simulink library "Contact_Forces_Lib"  (R2025b)
settings: Solver=ode45  StartTime=0.0  StopTime=10.0  RelTol=1e-3  EnableMultiTasking=on
undefined symbols (not defined in the file or in its folder): b_contact, custom_param_1, custom_param_2, Extr_Data_Ring, k_contact, l_cone, length_cylinder, length_tube, mu_kinetic, mu_static, pen_exponent, pen_full_damp_F, rad_s_cone, radius_cylinder, radius_tube, v_thr, X, Y, Z
libraries: nesl_utility x197, sm_lib x115, $bdroot x72, simulink x20, fl_lib x4
(part 5 of 12)

== system Contact_Forces_Lib/3D/Sphere to Tube Force ==
  Bus Creator1 : BusCreator  Inputs=3
  Check Active : Subsystem
  Demux : Subsystem
  External Force and Torque SphF : sm_lib/Forces and Torques/External Force and Torque  EnableForceX=on  EnableForceY=on  EnableForceZ=on  EnableForce=off  ForceResolutionFrame=AttachedFrame  EnableTorqueX=off  EnableTorqueY=off  EnableTorqueZ=off  EnableTorque=on  TorqueResolutionFrame=AttachedFrame
  External Force and Torque TubB : sm_lib/Forces and Torques/External Force and Torque  EnableForceX=on  EnableForceY=on  EnableForceZ=on  EnableForce=off  ForceResolutionFrame=AttachedFrame  EnableTorqueX=off  EnableTorqueY=off  EnableTorqueZ=off  EnableTorque=on  TorqueResolutionFrame=AttachedFrame
  Forces : Subsystem
  If1 : If
  Merge : Merge  InitialOutput=0  InputPortOffsets=0
  No Force : Subsystem
  Sensing : Subsystem
  Set Output : Subsystem
  Visual SphF : sm_lib/Body Elements/Spherical Solid  SphereRadius=radius_sphere  SphereRadiusUnits=m  ExportEntireGeometry=off  InertiaType=CalculateFromGeometry  BasedOnType=Density  Density=0  DensityUnits=kg/(m^3)  Mass=1  MassUnits=kg  CenterOfMass=[0 0 0]  CenterOfMassUnits=m  MomentsOfInertia=[1 1 1]  MomentsOfInertiaUnits=kg*m^2  ProductsOfInertia=[0 0 0]  ProductsOfInertiaUnits=kg*m^2  GraphicType=FromGeometry  MarkerShape=Sphere  MarkerSize=10  GraphicVisPropType=SimpleVisualProperties  GraphicDiffuseColor=vis_clr  GraphicOpacity=vis_opc*vis_opc_en  GraphicSpecularColor=[0.5 0.5 0.5 1.0]  GraphicAmbientColor=[0.15 0.15 0.15 1.0]  GraphicEmissiveColor=[0.0 0.0 0.0 1.0]  GraphicShininess=75  DoExposeReferenceFrame=on  SerializedFrames=<Frames/>
  Visual TubB Inner : sm_lib/Body Elements/Extruded Solid  ExtrusionType=General  PolygonNumSides=3  PolygonOuterRadius=1  PolygonOuterRadiusUnits=m  ExportEntireGeometry=off  ExtrusionCrossSection=Extr_Data_Ring(radius_tube-d_tube/2+vis_len_tubBx,radius_tube-d_tube/2,active_angle(1),active_angle(2))  ExtrusionCrossSectionUnits=m  ExportConvexHullGeometry=off  ExtrusionLength=l_tube  ExtrusionLengthUnits=m  InertiaType=CalculateFromGeometry  BasedOnType=Density  Density=0  DensityUnits=kg/(m^3)  Mass=1  MassUnits=kg  CenterOfMass=[0 0 0]  CenterOfMassUnits=m  MomentsOfInertia=[1 1 1]  MomentsOfInertiaUnits=kg*m^2  ProductsOfInertia=[0 0 0]  ProductsOfInertiaUnits=kg*m^2  GraphicType=FromGeometry  MarkerShape=Sphere  MarkerSize=10  GraphicVisPropType=SimpleVisualProperties  GraphicDiffuseColor=vis_clr  GraphicOpacity=vis_opc*vis_opc_en  GraphicSpecularColor=[0.5 0.5 0.5 1.0]  GraphicAmbientColor=[0.15 0.15 0.15 1.0]  GraphicEmissiveColor=[0.0 0.0 0.0 1.0]  GraphicShininess=75  DoExposeReferenceFrame=on  SerializedFrames=<Frames/>
  Visual TubB Outer : sm_lib/Body Elements/Extruded Solid  ExtrusionType=General  PolygonNumSides=3  PolygonOuterRadius=1  PolygonOuterRadiusUnits=m  ExportEntireGeometry=off  ExtrusionCrossSection=Extr_Data_Ring(radius_tube+d_tube/2,radius_tube+d_tube/2-vis_len_tubBx,active_angle(1),active_angle(2))  ExtrusionCrossSectionUnits=m  ExportConvexHullGeometry=off  ExtrusionLength=l_tube  ExtrusionLengthUnits=m  InertiaType=CalculateFromGeometry  BasedOnType=Density  Density=0  DensityUnits=kg/(m^3)  Mass=1  MassUnits=kg  CenterOfMass=[0 0 0]  CenterOfMassUnits=m  MomentsOfInertia=[1 1 1]  MomentsOfInertiaUnits=kg*m^2  ProductsOfInertia=[0 0 0]  ProductsOfInertiaUnits=kg*m^2  GraphicType=FromGeometry  MarkerShape=Sphere  MarkerSize=10  GraphicVisPropType=SimpleVisualProperties  GraphicDiffuseColor=vis_clr  GraphicOpacity=vis_opc*vis_opc_en  GraphicSpecularColor=[0.5 0.5 0.5 1.0]  GraphicAmbientColor=[0.15 0.15 0.15 1.0]  GraphicEmissiveColor=[0.0 0.0 0.0 1.0]  GraphicShininess=75  DoExposeReferenceFrame=on  SerializedFrames=<Frames/>
  SphF : PMIOPort  Tag=PMCPort  Side=Left
  TubB : PMIOPort  Tag=PMCPort  Port=2  Side=Right
  Out : Outport  VectorParamsAs1DForOutWhenUnconnected=off
  wires:
  Sensing/10(wyf) -> Forces/10(wyf)
  Sensing/9(wxf) -> Forces/9(wxf)
  Sensing/8(vzf) -> Forces/8(vzf)
  Sensing/1(z) -> Check Active/1(z), Forces/1(z)
  Merge/1 -> Demux/1(Frc)  "Total Force"
  Sensing/6(wzf) -> Forces/6(wzf)
  Sensing/3(vrad) -> Forces/3(vrad), Bus Creator1/2  "vrad"
  Sensing/4(azm) -> Check Active/2(azm), Forces/4(azm), Bus Creator1/3  "azm"
  If1/2 -> No Force/Action
  If1/1 -> Forces/Action
  No Force/1(F) -> Merge/1
  Forces/1(Frc) -> Merge/2
  Sensing/7(R) -> Forces/7(R)
  Sensing/2(rad) -> Forces/2(rad), Bus Creator1/1  "rad"
  Sensing/5(vazm) -> Forces/5(vazm)
  Forces/2(Out) -> Set Output/1(Frc)
  Bus Creator1/1 -> Set Output/3(FrameSep)  "Frame Sep"
  Set Output/1(Out) -> Out/1
  Check Active/1(En) -> Set Output/2(En), If1/1
  connections:
  Demux/RConn8 -- External Force and Torque TubB/LConn4
  Demux/RConn7 -- External Force and Torque TubB/LConn3
  Demux/RConn6 -- External Force and Torque TubB/LConn2
  Demux/RConn5 -- External Force and Torque TubB/LConn1
  Demux/RConn4 -- External Force and Torque SphF/LConn4
  Demux/RConn3 -- External Force and Torque SphF/LConn3
  Demux/RConn2 -- External Force and Torque SphF/LConn2
  Demux/RConn1 -- External Force and Torque SphF/LConn1
  External Force and Torque SphF/RConn1 -- Visual SphF/RConn1 -- SphF/RConn1 -- Sensing/LConn1
  Visual TubB Outer/RConn1 -- Visual TubB Inner/RConn1 -- TubB/RConn1 -- Sensing/LConn2 -- External Force and Torque TubB/RConn1

== system Contact_Forces_Lib/3D/Sphere to Tube Force Enabled ==
  In : Inport
  Bus Creator1 : BusCreator  Inputs=3
  Bus Selector1 : BusSelector  OutputSignals=Enable
  Check Active : Subsystem
  Demux : Subsystem
  External Force and Torque SphF : sm_lib/Forces and Torques/External Force and Torque  EnableForceX=on  EnableForceY=on  EnableForceZ=on  EnableForce=off  ForceResolutionFrame=AttachedFrame  EnableTorqueX=off  EnableTorqueY=off  EnableTorqueZ=off  EnableTorque=on  TorqueResolutionFrame=AttachedFrame
  External Force and Torque TubB : sm_lib/Forces and Torques/External Force and Torque  EnableForceX=on  EnableForceY=on  EnableForceZ=on  EnableForce=off  ForceResolutionFrame=AttachedFrame  EnableTorqueX=off  EnableTorqueY=off  EnableTorqueZ=off  EnableTorque=on  TorqueResolutionFrame=AttachedFrame
  Forces : Subsystem
  If1 : If  NumInputs=2  IfExpression=(u1 > 0 & u2>0)
  In1 : InportShadow
  Merge : Merge  InitialOutput=0  InputPortOffsets=0
  No Force : Subsystem
  Sensing : Subsystem
  Set Output : Subsystem
  Visual SphF : sm_lib/Body Elements/Spherical Solid  SphereRadius=radius_sphere  SphereRadiusUnits=m  ExportEntireGeometry=off  InertiaType=CalculateFromGeometry  BasedOnType=Density  Density=0  DensityUnits=kg/(m^3)  Mass=1  MassUnits=kg  CenterOfMass=[0 0 0]  CenterOfMassUnits=m  MomentsOfInertia=[1 1 1]  MomentsOfInertiaUnits=kg*m^2  ProductsOfInertia=[0 0 0]  ProductsOfInertiaUnits=kg*m^2  GraphicType=FromGeometry  MarkerShape=Sphere  MarkerSize=10  GraphicVisPropType=SimpleVisualProperties  GraphicDiffuseColor=vis_clr  GraphicOpacity=vis_opc*vis_opc_en  GraphicSpecularColor=[0.5 0.5 0.5 1.0]  GraphicAmbientColor=[0.15 0.15 0.15 1.0]  GraphicEmissiveColor=[0.0 0.0 0.0 1.0]  GraphicShininess=75  DoExposeReferenceFrame=on  SerializedFrames=<Frames/>
  Visual TubB Inner : sm_lib/Body Elements/Extruded Solid  ExtrusionType=General  PolygonNumSides=3  PolygonOuterRadius=1  PolygonOuterRadiusUnits=m  ExportEntireGeometry=off  ExtrusionCrossSection=Extr_Data_Ring(radius_tube-d_tube/2+vis_len_tubBx,radius_tube-d_tube/2,active_angle(1),active_angle(2))  ExtrusionCrossSectionUnits=m  ExportConvexHullGeometry=off  ExtrusionLength=l_tube  ExtrusionLengthUnits=m  InertiaType=CalculateFromGeometry  BasedOnType=Density  Density=0  DensityUnits=kg/(m^3)  Mass=1  MassUnits=kg  CenterOfMass=[0 0 0]  CenterOfMassUnits=m  MomentsOfInertia=[1 1 1]  MomentsOfInertiaUnits=kg*m^2  ProductsOfInertia=[0 0 0]  ProductsOfInertiaUnits=kg*m^2  GraphicType=FromGeometry  MarkerShape=Sphere  MarkerSize=10  GraphicVisPropType=SimpleVisualProperties  GraphicDiffuseColor=vis_clr  GraphicOpacity=vis_opc*vis_opc_en  GraphicSpecularColor=[0.5 0.5 0.5 1.0]  GraphicAmbientColor=[0.15 0.15 0.15 1.0]  GraphicEmissiveColor=[0.0 0.0 0.0 1.0]  GraphicShininess=75  DoExposeReferenceFrame=on  SerializedFrames=<Frames/>
  Visual TubB Outer : sm_lib/Body Elements/Extruded Solid  ExtrusionType=General  PolygonNumSides=3  PolygonOuterRadius=1  PolygonOuterRadiusUnits=m  ExportEntireGeometry=off  ExtrusionCrossSection=Extr_Data_Ring(radius_tube+d_tube/2,radius_tube+d_tube/2-vis_len_tubBx,active_angle(1),active_angle(2))  ExtrusionCrossSectionUnits=m  ExportConvexHullGeometry=off  ExtrusionLength=l_tube  ExtrusionLengthUnits=m  InertiaType=CalculateFromGeometry  BasedOnType=Density  Density=0  DensityUnits=kg/(m^3)  Mass=1  MassUnits=kg  CenterOfMass=[0 0 0]  CenterOfMassUnits=m  MomentsOfInertia=[1 1 1]  MomentsOfInertiaUnits=kg*m^2  ProductsOfInertia=[0 0 0]  ProductsOfInertiaUnits=kg*m^2  GraphicType=FromGeometry  MarkerShape=Sphere  MarkerSize=10  GraphicVisPropType=SimpleVisualProperties  GraphicDiffuseColor=vis_clr  GraphicOpacity=vis_opc*vis_opc_en  GraphicSpecularColor=[0.5 0.5 0.5 1.0]  GraphicAmbientColor=[0.15 0.15 0.15 1.0]  GraphicEmissiveColor=[0.0 0.0 0.0 1.0]  GraphicShininess=75  DoExposeReferenceFrame=on  SerializedFrames=<Frames/>
  SphF : PMIOPort  Tag=PMCPort  Side=Left
  TubB : PMIOPort  Tag=PMCPort  Port=2  Side=Right
  Out : Outport  VectorParamsAs1DForOutWhenUnconnected=off
  wires:
  In1/1 -> Sensing/1(In)
  Bus Selector1/1 -> If1/1  "<Enable>"
  In/1 -> Bus Selector1/1
  Sensing/10(wyf) -> Forces/10(wyf)
  Sensing/9(wxf) -> Forces/9(wxf)
  Sensing/8(vzf) -> Forces/8(vzf)
  Sensing/1(z) -> Check Active/1(z), Forces/1(z)
  Merge/1 -> Demux/1(Frc)  "Total Force"
  Sensing/6(wzf) -> Forces/6(wzf)
  Sensing/3(vrad) -> Forces/3(vrad), Bus Creator1/2  "vrad"
  Sensing/4(azm) -> Check Active/2(azm), Forces/4(azm), Bus Creator1/3  "azm"
  If1/2 -> No Force/Action
  If1/1 -> Forces/Action
  No Force/1(F) -> Merge/1
  Forces/1(Frc) -> Merge/2
  Sensing/7(R) -> Forces/7(R)
  Sensing/2(rad) -> Forces/2(rad), Bus Creator1/1  "rad"
  Sensing/5(vazm) -> Forces/5(vazm)
  Forces/2(Out) -> Set Output/1(Frc)
  Bus Creator1/1 -> Set Output/3(FrameSep)  "Frame Sep"
  Set Output/1(Out) -> Out/1
  Check Active/1(En) -> If1/2, Set Output/2(En)
  connections:
  Demux/RConn8 -- External Force and Torque TubB/LConn4
  Demux/RConn7 -- External Force and Torque TubB/LConn3
  Demux/RConn6 -- External Force and Torque TubB/LConn2
  Demux/RConn5 -- External Force and Torque TubB/LConn1
  Demux/RConn4 -- External Force and Torque SphF/LConn4
  Demux/RConn3 -- External Force and Torque SphF/LConn3
  Demux/RConn2 -- External Force and Torque SphF/LConn2
  Demux/RConn1 -- External Force and Torque SphF/LConn1
  SphF/RConn1 -- External Force and Torque SphF/RConn1 -- Visual SphF/RConn1 -- Sensing/LConn1
  Visual TubB Outer/RConn1 -- Visual TubB Inner/RConn1 -- Sensing/LConn2 -- TubB/RConn1 -- External Force and Torque TubB/RConn1

== system Contact_Forces_Lib/Constraints/Cam Roller Constraint ==
  Cam : sm_lib/Body Elements/Extruded Solid  ExtrusionType=General  PolygonNumSides=3  PolygonOuterRadius=1  PolygonOuterRadiusUnits=m  ExportEntireGeometry=off  ExtrusionCrossSection=cam_extr_data  ExtrusionCrossSectionUnits=m  ExportConvexHullGeometry=off  ExtrusionLength=cam_thk  ExtrusionLengthUnits=m  InertiaType=CalculateFromGeometry  BasedOnType=Density  Density=cam_rho  DensityUnits=kg/m^3  Mass=1  MassUnits=kg  CenterOfMass=[0 0 0]  CenterOfMassUnits=m  MomentsOfInertia=[1 1 1]  MomentsOfInertiaUnits=kg*m^2  ProductsOfInertia=[1 1 1]  ProductsOfInertiaUnits=kg*m^2  GraphicType=FromGeometry  MarkerShape=Sphere  MarkerSize=10  GraphicVisPropType=SimpleVisualProperties  GraphicDiffuseColor=cam_clr  GraphicOpacity=cam_opc  GraphicSpecularColor=[0.5 0.5 0.5 1.0]  GraphicAmbientColor=[0.15 0.15 0.15 1.0]  GraphicEmissiveColor=[0.0 0.0 0.0 1.0]  GraphicShininess=75  DoExposeReferenceFrame=on  SerializedFrames=<Frames/>
  Point on Curve Constraint : sm_lib/Constraints/Point on Curve Constraint  WrenchDir=FollowerOnBase  WrenchFrame=BaseFrame  SenseForce=off  SenseTorque=off
  Roller : sm_lib/Body Elements/Cylindrical Solid  CylinderRadius=roller_rad  CylinderRadiusUnits=m  CylinderLength=roller_thk  CylinderLengthUnits=m  ExportEntireGeometry=off  InertiaType=CalculateFromGeometry  BasedOnType=Density  Density=roller_rho  DensityUnits=kg/m^3  Mass=1  MassUnits=kg  CenterOfMass=[0 0 0]  CenterOfMassUnits=m  MomentsOfInertia=[1 1 1]  MomentsOfInertiaUnits=kg*m^2  ProductsOfInertia=[1 1 1]  ProductsOfInertiaUnits=kg*m^2  GraphicType=FromGeometry  MarkerShape=Sphere  MarkerSize=10  GraphicVisPropType=SimpleVisualProperties  GraphicDiffuseColor=roller_clr  GraphicOpacity=roller_opc  GraphicSpecularColor=[0.5 0.5 0.5 1.0]  GraphicAmbientColor=[0.15 0.15 0.15 1.0]  GraphicEmissiveColor=[0.0 0.0 0.0 1.0]  GraphicShininess=75  DoExposeReferenceFrame=on  SerializedFrames=<Frames/>
  Spline : sm_lib/Curves and Surfaces/Spline  DataPoints=roller_curve  DataPointsUnits=m  EndConditionType=Closed  GraphicType=FromGeometry  MarkerShape=Sphere  MarkerSize=10  GraphicVisPropType=SimpleVisualProperties  GraphicDiffuseColor=roller_curve_clr  GraphicOpacity=roller_curve_opc  GraphicSpecularColor=[0.5 0.5 0.5 1.0]  GraphicAmbientColor=[0.15 0.15 0.15 1.0]  GraphicEmissiveColor=[0.0 0.0 0.0 1.0]  GraphicShininess=75
  C : PMIOPort  Side=Right
  R : PMIOPort  Port=2  Side=Left
  connections:
  C/RConn1 -- Cam/RConn1 -- Spline/LConn1
  Spline/RConn1 -- Point on Curve Constraint/LConn1
  Point on Curve Constraint/RConn1 -- R/RConn1 -- Roller/RConn1

== system Contact_Forces_Lib/Force Law/Custom ==
  note: Implement your own custom force law in this subsystem.
      | To use it in the contact force models,
      | set the parameter "Force Law" to "Custom".
  Pen : Inport
  Pen Vel : Inport  Port=2
  Abs : Abs  ZeroCross=off  SaturateOnIntegerOverflow=off
  Gain1 : Gain  Gain=k_pen  Multiplication=Matrix(K*u)  SaturateOnIntegerOverflow=on  OutDataTypeStr=Inherit: Same as input  ParamDataTypeStr=Inherit: Same as input
  Gain2 : Gain  Gain=-b_penvel  Multiplication=Matrix(K*u)  SaturateOnIntegerOverflow=on  OutDataTypeStr=Inherit: Same as input  ParamDataTypeStr=Inherit: Same as input
  Product : Product  RndMeth=Zero
  Saturation : Saturate  UpperLimit=Inf  LowerLimit=0  ZeroCross=off
  Sign : Signum  ZeroCross=off
  Spr F : Outport  VectorParamsAs1DForOutWhenUnconnected=off
  Damp F : Outport  Port=2  VectorParamsAs1DForOutWhenUnconnected=off
  wires:
  Gain1/1 -> Spr F/1  "Stiffness_Force"
  Gain2/1 -> Product/2  "Damping_Force"
  Pen Vel/1 -> Saturation/1  "Pen Vel"
  Sign/1 -> Abs/1
  Product/1 -> Damp F/1  "Damping_Force"
  Abs/1 -> Product/1  "Damping_Force_Enable"
  Pen/1 -> Gain1/1, Sign/1  "Penetration"
  Saturation/1 -> Gain2/1

== system Contact_Forces_Lib/Force Law/Linear ==
  Pen : Inport
  Pen Vel : Inport  Port=2
  Abs : Abs  ZeroCross=off  SaturateOnIntegerOverflow=off
  Gain1 : Gain  Gain=k_pen  Multiplication=Matrix(K*u)  SaturateOnIntegerOverflow=on  OutDataTypeStr=Inherit: Same as input  ParamDataTypeStr=Inherit: Same as input
  Gain2 : Gain  Gain=-b_penvel  Multiplication=Matrix(K*u)  SaturateOnIntegerOverflow=on  OutDataTypeStr=Inherit: Same as input  ParamDataTypeStr=Inherit: Same as input
  Product : Product  RndMeth=Zero
  Saturation : Saturate  UpperLimit=Inf  LowerLimit=0  ZeroCross=off
  Sign : Signum  ZeroCross=off
  Spr F : Outport  VectorParamsAs1DForOutWhenUnconnected=off
  Damp F : Outport  Port=2  VectorParamsAs1DForOutWhenUnconnected=off
  wires:
  Gain1/1 -> Spr F/1  "Stiffness_Force"
  Gain2/1 -> Product/2  "Damping_Force"
  Pen Vel/1 -> Saturation/1  "Pen Vel"
  Sign/1 -> Abs/1
  Product/1 -> Damp F/1  "Damping_Force"
  Abs/1 -> Product/1  "Damping_Force_Enable"
  Pen/1 -> Gain1/1, Sign/1  "Penetration"
  Saturation/1 -> Gain2/1

== system Contact_Forces_Lib/Force Law/Nonlinear ==
  Pen : Inport
  Pen Vel : Inport  Port=2
  Constant : Constant  Value=pen_exp
  Gain1 : Gain  Gain=k_pen  Multiplication=Matrix(K*u)  SaturateOnIntegerOverflow=on  OutDataTypeStr=Inherit: Same as input  ParamDataTypeStr=Inherit: Same as input
  Gain2 : Gain  Gain=-b_penvel  Multiplication=Matrix(K*u)  SaturateOnIntegerOverflow=on  OutDataTypeStr=Inherit: Same as input  ParamDataTypeStr=Inherit: Same as input
  Math Function : Math  Operator=pow  SignedPower=on
  Product1 : Product  RndMeth=Zero
  Saturation : Saturate  UpperLimit=Inf  LowerLimit=0  ZeroCross=off
  Smoothstep : Subsystem  mask{min_out=0, max_out=1, step_start=0, step_finish=pen_full_damping}
      mask prompts: min_out "Minimum output"; max_out "Maximum output"; step_start "Start Step"; step_finish "Finish Step"
  Spr F : Outport  VectorParamsAs1DForOutWhenUnconnected=off
  Damp F : Outport  Port=2  VectorParamsAs1DForOutWhenUnconnected=off
  wires:
  Gain1/1 -> Spr F/1  "Stiffness_Force"
  Pen Vel/1 -> Saturation/1  "Penetration_Velocity"
  Pen/1 -> Smoothstep/1(In1), Math Function/1  "Penetration"
  Math Function/1 -> Gain1/1
  Constant/1 -> Math Function/2
  Gain2/1 -> Product1/2  "Damping_Force"
  Smoothstep/1(Out1) -> Product1/1  "Damping_Enable"
  Product1/1 -> Damp F/1
  Saturation/1 -> Gain2/1

== system Contact_Forces_Lib/Friction Law/None ==
  Fn : Inport
  v : Inport  Port=2
  Constant : Constant  Value=0
  Terminator : Terminator
  Terminator1 : Terminator
  Ff : Outport  VectorParamsAs1DForOutWhenUnconnected=off
  wires:
  Fn/1 -> Terminator1/1  "Normal_Force"
  v/1 -> Terminator/1  "Velocity"
  Constant/1 -> Ff/1  "Friction_Force"

== system Contact_Forces_Lib/Friction Law/Stick-Slip C  ==
  Fn : Inport
  v : Inport  Port=2
  Coefficient of Friction vs Velocity : Lookup_n-D  NumberOfTableDimensions=1  BreakpointsForDimension1=[-3 -1.5 -1 1 1.5 3]*vth  Table="[-muk -muk -mus mus  muk muk]"  InternalRulePriority=Speed
  Gain2 : Gain  Multiplication=Matrix(K*u)  SaturateOnIntegerOverflow=on  OutDataTypeStr=Inherit: Same as input  ParamDataTypeStr=Inherit: Same as input
  Product : Product  RndMeth=Zero
  Ff : Outport  VectorParamsAs1DForOutWhenUnconnected=off
  wires:
  Gain2/1 -> Ff/1  "Friction_Force"
  Product/1 -> Gain2/1
  v/1 -> Coefficient of Friction vs Velocity/1  "Velocity"
  Coefficient of Friction vs Velocity/1 -> Product/1
  Fn/1 -> Product/2  "Normal_Force"

== system Contact_Forces_Lib/Friction Utilities/Stick-Slip Friction 1D ==
  Abs : Abs  ZeroCross=off  SaturateOnIntegerOverflow=off
  Gain : Gain  Gain=-1
  Lag Filter : Subsystem  mask(First-order lag supporting vector signals){b=filt_const, x_initial=0}
      mask prompts: b "Filter time constant"; x_initial "Initial output"
      mask help: Models a lag of the form 1/(b*s+1) where s is the Laplace operator.
  PS-Simulink Converter : nesl_utility/PS-Simulink Converter  PhysicalDomain=network_engine_domain  SubClassName=ps_output  LeftPortType=input  RightPortType=output  PseudoPeriodic=off  Frequencies=[]  VectorFormat=1-D array  Unit=1  AffineConversion=off
  PS-Simulink Converter1 : nesl_utility/PS-Simulink Converter  PhysicalDomain=network_engine_domain  SubClassName=ps_output  LeftPortType=input  RightPortType=output  PseudoPeriodic=off  Frequencies=[]  VectorFormat=1-D array  Unit=1  AffineConversion=off
  Product : $bdroot/Friction Utilities/Utilities/Product  SystemSampleTime=-1  LabelModeActiveChoice=FcConst  VariantActivationTime=update diagram  EmptyChoice=off  PassThrough=off  PassThroughVariantControl=(default)  EmptyChoiceVariantControl=(default)  AllowFlexibleInterface=on  Latency=0  AutoFrameSizeCalculation=off
  Selector : Selector  InputPortWidth=3  IndexOptions=Index vector (dialog)  Indices=[1]  OutputSizes=1
  Simulink-PS Converter1 : nesl_utility/Simulink-PS Converter  PhysicalDomain=network_engine_domain  SubClassName=ps_input  LeftPortType=input  RightPortType=output  PseudoPeriodic=off  Frequencies=[]  NoiseDistribution=none  NoiseParameters=[]  Unit=1  AffineConversion=off  FilteringAndDerivatives=zero  SimscapeFilterOrder=2  InputFilterTimeConstant=0.005  UdotUserProvided=1
  "Stick-Slip C " : $bdroot/Friction Law/Stick-Slip C   VariantControl=Stick_Slip_C  muk=mu_kinetic  mus=mu_static  vth=vel_th
  Vectorize : Gain  Gain=[1 1 1]
  f : PMIOPort  Side=Right
  Fc : PMIOPort  Port=2  Side=Left
  v : PMIOPort  Port=3  Side=Left
  wires:
  Gain/1 -> "Stick-Slip C "/1
  Abs/1 -> Gain/1
  Vectorize/1 -> Selector/1
  PS-Simulink Converter/1 -> "Stick-Slip C "/2
  PS-Simulink Converter1/1 -> Vectorize/1
  "Stick-Slip C "/1 -> Lag Filter/1(In)
  Selector/1 -> Abs/1
  Lag Filter/1(Out) -> Simulink-PS Converter1/1
  connections:
  v/RConn1 -- PS-Simulink Converter/LConn1 -- Product/RConn2
  Fc/RConn1 -- PS-Simulink Converter1/LConn1 -- Product/RConn1
  Simulink-PS Converter1/RConn1 -- f/RConn1

== system Contact_Forces_Lib/Friction Utilities/Utilities ==
  Product : Subsystem  Variant=on  VariantControlMode=label  LabelModeActiveChoice=FcConst

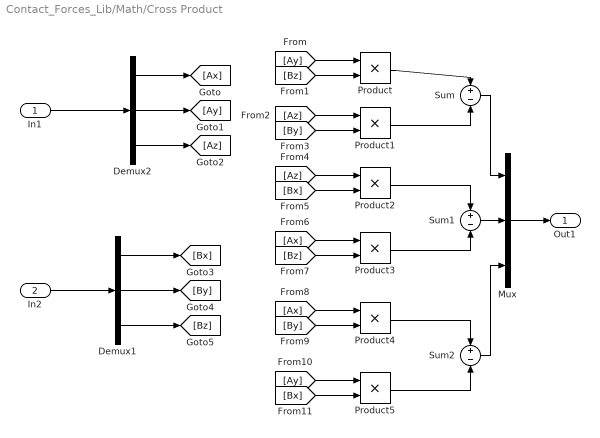
== system Contact_Forces_Lib/Math/Cross Product ==
  In1 : Inport
  In2 : Inport  Port=2
  Demux1 : Demux  Outputs=3
  Demux2 : Demux  Outputs=3
  Mux : Mux  Inputs=3
  Product{,1..5} (6 alike) : Product
  Sum : Sum  Inputs=+|-
  Sum1 : Sum  Inputs=+|-
  Sum2 : Sum  Inputs=+|-
  Out1 : Outport  VectorParamsAs1DForOutWhenUnconnected=off
  wires:
  [Bx] -> Product5/2
  [Ay] -> Product5/1
  [By] -> Product4/2
  [Ax] -> Product4/1
  [Bz] -> Product3/2
  [Ax] -> Product3/1
  [Bx] -> Product2/2
  [Az] -> Product2/1
  [By] -> Product1/2
  [Az] -> Product1/1
  [Bz] -> Product/2
  [Ay] -> Product/1
  Demux1/3 -> [Bz]
  Demux1/2 -> [By]
  Demux1/1 -> [Bx]
  Demux2/3 -> [Az]
  Demux2/2 -> [Ay]
  Demux2/1 -> [Ax]
  In1/1 -> Demux2/1
  Sum2/1 -> Mux/3
  Sum/1 -> Mux/1
  Sum1/1 -> Mux/2
  Product5/1 -> Sum2/2
  Product4/1 -> Sum2/1
  Product3/1 -> Sum1/2
  Product2/1 -> Sum1/1
  Product/1 -> Sum/1
  Product1/1 -> Sum/2
  Mux/1 -> Out1/1
  In2/1 -> Demux1/1

== system Contact_Forces_Lib/Other Forces/Attraction Force ==
  Pen : Inport
  Pen Vel : Inport  Port=2
  Abs : Abs  SaturateOnIntegerOverflow=off
  Dead Zone Center : DeadZone  LowerValue=-inf  UpperValue=0
  Dead Zone Radius : Constant  Value=max_sep*deadzone
  Enable Stiffness Force : Product  RndMeth=Zero
  Gain1 : Gain  Gain=k_pen  Multiplication=Matrix(K*u)  SaturateOnIntegerOverflow=on  OutDataTypeStr=Inherit: Same as input  ParamDataTypeStr=Inherit: Same as input
  Gain2 : Gain  Gain=-b_penvel  Multiplication=Matrix(K*u)  SaturateOnIntegerOverflow=on  OutDataTypeStr=Inherit: Same as input  ParamDataTypeStr=Inherit: Same as input
  Gain3 : Gain  Gain=1e2  Multiplication=Matrix(K*u)  SaturateOnIntegerOverflow=on  OutDataTypeStr=Inherit: Same as input  ParamDataTypeStr=Inherit: Same as input
  Product : Product  RndMeth=Zero
  Sum1 : Sum  Inputs=|-+
  Spr Force : Outport  VectorParamsAs1DForOutWhenUnconnected=off
  Damp Force : Outport  Port=2  VectorParamsAs1DForOutWhenUnconnected=off
  wires:
  Enable Stiffness Force/1 -> Spr Force/1
  Gain1/1 -> Enable Stiffness Force/1  "Stiffness_Force"
  Dead Zone Center/1 -> Enable Stiffness Force/2
  Sum1/1 -> Dead Zone Center/1
  Dead Zone Radius/1 -> Sum1/2
  Pen/1 -> Sum1/1, Gain1/1, Gain3/1  "Penetration"
  Abs/1 -> Product/1  "Damping_Force_Enable"
  Product/1 -> Damp Force/1  "Damping_Force"
  Gain3/1 -> Abs/1
  Pen Vel/1 -> Gain2/1  "Penetration_Velocity"
  Gain2/1 -> Product/2  "Damping_Force"

== system Contact_Forces_Lib/2D/Circle to Circle Force/Calculate Penetration ==
  rad : Inport
  vrad : Inport  Port=2
  Constant : Constant  Value=cirF_rad+cirB_rad
  Dead Zone : DeadZone  LowerValue=-inf  UpperValue=0
  Gain2 : Gain  Gain=-1
  Sum1 : Sum  Inputs=+-
  Pen : Outport  VectorParamsAs1DForOutWhenUnconnected=off
  Pen Vel : Outport  Port=2  VectorParamsAs1DForOutWhenUnconnected=off
  wires:
  rad/1 -> Sum1/2
  Constant/1 -> Sum1/1
  Sum1/1 -> Dead Zone/1
  Dead Zone/1 -> Pen/1
  Gain2/1 -> Pen Vel/1
  vrad/1 -> Gain2/1

== system Contact_Forces_Lib/2D/Circle to Circle Force/Ff ==
  Fn : Inport
  azm : Inport  Port=2
  Pen : Inport  Port=3
  rad : Inport  Port=4
  R : Inport  Port=5
  wz : Inport  Port=6
  vazm : Inport  Port=7
  "Calculate vRel at CP " : Subsystem
  Friction Law : $bdroot/Friction Law  SystemSampleTime=-1  LabelModeActiveChoice=None  VariantActivationTime=update diagram  EmptyChoice=off  PassThrough=off  PassThroughVariantControl=(default)  EmptyChoiceVariantControl=(default)  AllowFlexibleInterface=on  Latency=0  AutoFrameSizeCalculation=off
  Resolve Ff : Subsystem
  FxCirF : Outport  VectorParamsAs1DForOutWhenUnconnected=off
  FyCirF : Outport  Port=2  VectorParamsAs1DForOutWhenUnconnected=off
  FxCirB : Outport  Port=3  VectorParamsAs1DForOutWhenUnconnected=off
  FyCirB : Outport  Port=4  VectorParamsAs1DForOutWhenUnconnected=off
  TzCirF : Outport  Port=5  VectorParamsAs1DForOutWhenUnconnected=off
  TzCirB : Outport  Port=6  VectorParamsAs1DForOutWhenUnconnected=off
  Ff : Outport  Port=7  VectorParamsAs1DForOutWhenUnconnected=off
  wires:
  R/1 -> Resolve Ff/2(R)
  azm/1 -> Resolve Ff/3(azm)
  Pen/1 -> "Calculate vRel at CP "/2(Pen)
  Fn/1 -> Friction Law/1
  rad/1 -> "Calculate vRel at CP "/1(rad)
  "Calculate vRel at CP "/1(vRelCP) -> Friction Law/2
  Friction Law/1 -> Ff/1, Resolve Ff/1(Ff)
  Resolve Ff/4(FxCirF) -> FxCirF/1
  Resolve Ff/3(FyCirF) -> FyCirF/1
  Resolve Ff/1(FxCirB) -> FxCirB/1
  Resolve Ff/2(FyCirB) -> FyCirB/1
  Resolve Ff/5(TzCirF) -> TzCirF/1
  Resolve Ff/6(TzCirB) -> TzCirB/1
  wz/1 -> "Calculate vRel at CP "/3(wz)
  vazm/1 -> "Calculate vRel at CP "/4(vazm)
  "Calculate vRel at CP "/2(rCirFtoCP) -> Resolve Ff/4(rCirFtoCP)
  "Calculate vRel at CP "/3(rCirBtoCP) -> Resolve Ff/5(rCirBtoCP)

== system Contact_Forces_Lib/2D/Circle to Circle Force/Fn ==
  note: Resolve Normal Force in
      | Circle F reference frame
  note: Resolve Normal Force in
      | Circle B reference frame
  Fn : Inport
  R : Inport  Port=2
  azm : Inport  Port=3
  Fn in CirB : Subsystem
  Fn in CirF : Subsystem
  FxCirF : Outport  VectorParamsAs1DForOutWhenUnconnected=off
  FyCirF : Outport  Port=2  VectorParamsAs1DForOutWhenUnconnected=off
  FxCirB : Outport  Port=3  VectorParamsAs1DForOutWhenUnconnected=off
  FyCirB : Outport  Port=4  VectorParamsAs1DForOutWhenUnconnected=off
  wires:
  Fn in CirF/2(FxCirF) -> FxCirF/1
  Fn in CirF/1(FyCirF) -> FyCirF/1
  R/1 -> Fn in CirF/1(R)
  azm/1 -> Fn in CirB/2(azm)
  Fn/1 -> Fn in CirB/1(Fn)
  Fn in CirB/2(FyCirB) -> FyCirB/1, Fn in CirF/3(FyCirB)
  Fn in CirB/1(FxCirB) -> Fn in CirF/2(FxCirB), FxCirB/1

== system Contact_Forces_Lib/2D/Circle to Circle Force/Sensing ==
  PS-Simulink Converter1 : nesl_utility/PS-Simulink Converter  PhysicalDomain=network_engine_domain  SubClassName=ps_output  LeftPortType=input  RightPortType=output  PseudoPeriodic=off  Frequencies=[]  VectorFormat=1-D array  Unit=deg  AffineConversion=off
  PS-Simulink Converter{4..6,8..9} (5 alike) : nesl_utility/PS-Simulink Converter  PhysicalDomain=network_engine_domain  SubClassName=ps_output  LeftPortType=input  RightPortType=output  PseudoPeriodic=off  Frequencies=[]  VectorFormat=1-D array  Unit=1  AffineConversion=off
  Selector : Selector  NumberOfDimensions=2  InputPortWidth=3  IndexOptions=Index vector (dialog),Index vector (dialog)  Indices=[1,2],[1,2]  OutputSizes=1,1
  Transform Sensor Base : sm_lib/Frames and Transforms/Transform Sensor  MeasurementFrame=Base  RotationSequence=XYX  SenseAngle=off  SenseAxis=off  SenseQ=off  SenseR=on  SenseRotationSequence=off  SenseOmegaX=off  SenseOmegaY=off  SenseOmegaZ=on  SenseOmega=off  SenseQDot=off  SenseRDot=off  SenseRotationSequenceDot=off  SenseAlphaX=off  SenseAlphaY=off  SenseAlphaZ=off  SenseAlpha=off  SenseQDDot=off  SenseRDDot=off  SenseX=off  SenseY=off  SenseZ=off  SenseXYZ=off  SenseRad=on  SenseAzim=on  SenseDist=off  SenseInc=off  SenseXDot=off  SenseYDot=off  SenseZDot=off  SenseXYZDot=off  SenseRadDot=on  SenseAzimDot=on  SenseDistDot=off  SenseIncDot=off  SenseXDDot=off  SenseYDDot=off  SenseZDDot=off  SenseXYZDDot=off  SenseRadDDot=off  SenseAzimDDot=off  SenseDistDDot=off  SenseIncDDot=off
  F : PMIOPort  Side=Left
  B : PMIOPort  Port=2  Side=Left
  rad : Outport  VectorParamsAs1DForOutWhenUnconnected=off
  vrad : Outport  Port=2  VectorParamsAs1DForOutWhenUnconnected=off
  azm : Outport  Port=3  VectorParamsAs1DForOutWhenUnconnected=off
  R : Outport  Port=4  VectorParamsAs1DForOutWhenUnconnected=off
  wz : Outport  Port=5  VectorParamsAs1DForOutWhenUnconnected=off
  vazm : Outport  Port=6  VectorParamsAs1DForOutWhenUnconnected=off
  wires:
  PS-Simulink Converter1/1 -> azm/1
  PS-Simulink Converter5/1 -> rad/1
  PS-Simulink Converter4/1 -> vrad/1
  Selector/1 -> R/1
  PS-Simulink Converter6/1 -> Selector/1
  PS-Simulink Converter8/1 -> wz/1
  PS-Simulink Converter9/1 -> vazm/1
  connections:
  PS-Simulink Converter4/LConn1 -- Transform Sensor Base/RConn6
  PS-Simulink Converter5/LConn1 -- Transform Sensor Base/RConn4
  PS-Simulink Converter1/LConn1 -- Transform Sensor Base/RConn5
  PS-Simulink Converter6/LConn1 -- Transform Sensor Base/RConn2
  Transform Sensor Base/LConn1 -- B/RConn1
  Transform Sensor Base/RConn1 -- F/RConn1
  PS-Simulink Converter8/LConn1 -- Transform Sensor Base/RConn3
  PS-Simulink Converter9/LConn1 -- Transform Sensor Base/RConn7

== system Contact_Forces_Lib/2D/Circle to Circle Force/Sum ==
  FnxCirF : Inport
  FnyCirF : Inport  Port=2
  FnxCirB : Inport  Port=3
  FnyCirB : Inport  Port=4
  FfxCirF : Inport  Port=5
  FfyCirF : Inport  Port=6
  FfxCirB : Inport  Port=7
  FfyCirB : Inport  Port=8
  TzCirF : Inport  Port=9
  TzCirB : Inport  Port=10
  Simulink-PS Converter{,3..7} (6 alike) : nesl_utility/Simulink-PS Converter  PhysicalDomain=network_engine_domain  SubClassName=ps_input  LeftPortType=input  RightPortType=output  PseudoPeriodic=off  Frequencies=[]  NoiseDistribution=none  NoiseParameters=[]  Unit=1  AffineConversion=off  FilteringAndDerivatives=zero  SimscapeFilterOrder=1  InputFilterTimeConstant=0.005  UdotUserProvided=[]
  Sum{2..5} (4 alike) : Sum
  FxF : PMIOPort  Side=Right
  FyF : PMIOPort  Port=2  Side=Right
  TzF : PMIOPort  Port=3  Side=Right
  FxB : PMIOPort  Port=4  Side=Right
  FyB : PMIOPort  Port=5  Side=Right
  TzB : PMIOPort  Port=6  Side=Right
  wires:
  FfxCirF/1 -> Sum4/2
  FfyCirF/1 -> Sum2/2
  FfyCirB/1 -> Sum5/2
  FfxCirB/1 -> Sum3/2
  TzCirF/1 -> Simulink-PS Converter6/1
  TzCirB/1 -> Simulink-PS Converter7/1
  FnxCirF/1 -> Sum4/1
  FnyCirF/1 -> Sum2/1
  FnxCirB/1 -> Sum3/1
  FnyCirB/1 -> Sum5/1
  Sum4/1 -> Simulink-PS Converter/1
  Sum2/1 -> Simulink-PS Converter3/1
  Sum3/1 -> Simulink-PS Converter4/1
  Sum5/1 -> Simulink-PS Converter5/1
  connections:
  Simulink-PS Converter/RConn1 -- FxF/RConn1
  Simulink-PS Converter3/RConn1 -- FyF/RConn1
  Simulink-PS Converter4/RConn1 -- FxB/RConn1
  Simulink-PS Converter5/RConn1 -- FyB/RConn1
  Simulink-PS Converter6/RConn1 -- TzF/RConn1
  Simulink-PS Converter7/RConn1 -- TzB/RConn1

== system Contact_Forces_Lib/2D/Circle to Circle Force Enabled/Calculate Penetration ==
  rad : Inport
  vrad : Inport  Port=2
  Constant : Constant  Value=cirF_rad+cirB_rad
  Dead Zone : DeadZone  LowerValue=-inf  UpperValue=0
  Gain2 : Gain  Gain=-1
  Sum1 : Sum  Inputs=+-
  Pen : Outport  VectorParamsAs1DForOutWhenUnconnected=off
  Pen Vel : Outport  Port=2  VectorParamsAs1DForOutWhenUnconnected=off
  wires:
  vrad/1 -> Gain2/1
  Gain2/1 -> Pen Vel/1
  Dead Zone/1 -> Pen/1
  Sum1/1 -> Dead Zone/1
  Constant/1 -> Sum1/1
  rad/1 -> Sum1/2

== system Contact_Forces_Lib/2D/Circle to Circle Force Enabled/Ff ==
  Fn : Inport
  azm : Inport  Port=2
  Pen : Inport  Port=3
  rad : Inport  Port=4
  R : Inport  Port=5
  wz : Inport  Port=6
  vazm : Inport  Port=7
  "Calculate vRel at CP " : Subsystem
  Friction Law : $bdroot/Friction Law  SystemSampleTime=-1  LabelModeActiveChoice=None  VariantActivationTime=update diagram  EmptyChoice=off  PassThrough=off  PassThroughVariantControl=(default)  EmptyChoiceVariantControl=(default)  AllowFlexibleInterface=on  Latency=0  AutoFrameSizeCalculation=off
  Resolve Ff : Subsystem
  FxCirF : Outport  VectorParamsAs1DForOutWhenUnconnected=off
  FyCirF : Outport  Port=2  VectorParamsAs1DForOutWhenUnconnected=off
  FxCirB : Outport  Port=3  VectorParamsAs1DForOutWhenUnconnected=off
  FyCirB : Outport  Port=4  VectorParamsAs1DForOutWhenUnconnected=off
  TzCirF : Outport  Port=5  VectorParamsAs1DForOutWhenUnconnected=off
  TzCirB : Outport  Port=6  VectorParamsAs1DForOutWhenUnconnected=off
  Ff : Outport  Port=7  VectorParamsAs1DForOutWhenUnconnected=off
  wires:
  "Calculate vRel at CP "/3(rCirBtoCP) -> Resolve Ff/5(rCirBtoCP)
  "Calculate vRel at CP "/2(rCirFtoCP) -> Resolve Ff/4(rCirFtoCP)
  vazm/1 -> "Calculate vRel at CP "/4(vazm)
  wz/1 -> "Calculate vRel at CP "/3(wz)
  Resolve Ff/6(TzCirB) -> TzCirB/1
  Resolve Ff/5(TzCirF) -> TzCirF/1
  Resolve Ff/2(FyCirB) -> FyCirB/1
  Resolve Ff/1(FxCirB) -> FxCirB/1
  Resolve Ff/3(FyCirF) -> FyCirF/1
  Resolve Ff/4(FxCirF) -> FxCirF/1
  Friction Law/1 -> Resolve Ff/1(Ff), Ff/1
  "Calculate vRel at CP "/1(vRelCP) -> Friction Law/2
  rad/1 -> "Calculate vRel at CP "/1(rad)
  Fn/1 -> Friction Law/1
  Pen/1 -> "Calculate vRel at CP "/2(Pen)
  azm/1 -> Resolve Ff/3(azm)
  R/1 -> Resolve Ff/2(R)

== system Contact_Forces_Lib/2D/Circle to Circle Force Enabled/Fn ==
  note: Resolve Normal Force in
      | Circle B reference frame
  note: Resolve Normal Force in
      | Circle F reference frame
  Fn : Inport
  R : Inport  Port=2
  azm : Inport  Port=3
  Fn in CirB : Subsystem
  Fn in CirF : Subsystem
  FxCirF : Outport  VectorParamsAs1DForOutWhenUnconnected=off
  FyCirF : Outport  Port=2  VectorParamsAs1DForOutWhenUnconnected=off
  FxCirB : Outport  Port=3  VectorParamsAs1DForOutWhenUnconnected=off
  FyCirB : Outport  Port=4  VectorParamsAs1DForOutWhenUnconnected=off
  wires:
  Fn in CirB/1(FxCirB) -> FxCirB/1, Fn in CirF/2(FxCirB)
  Fn in CirB/2(FyCirB) -> Fn in CirF/3(FyCirB), FyCirB/1
  Fn/1 -> Fn in CirB/1(Fn)
  azm/1 -> Fn in CirB/2(azm)
  R/1 -> Fn in CirF/1(R)
  Fn in CirF/1(FyCirF) -> FyCirF/1
  Fn in CirF/2(FxCirF) -> FxCirF/1

== system Contact_Forces_Lib/2D/Circle to Circle Force Enabled/Sensing ==
  PS-Simulink Converter1 : nesl_utility/PS-Simulink Converter  PhysicalDomain=network_engine_domain  SubClassName=ps_output  LeftPortType=input  RightPortType=output  PseudoPeriodic=off  Frequencies=[]  VectorFormat=1-D array  Unit=deg  AffineConversion=off
  PS-Simulink Converter{4..6,8..9} (5 alike) : nesl_utility/PS-Simulink Converter  PhysicalDomain=network_engine_domain  SubClassName=ps_output  LeftPortType=input  RightPortType=output  PseudoPeriodic=off  Frequencies=[]  VectorFormat=1-D array  Unit=1  AffineConversion=off
  Selector : Selector  NumberOfDimensions=2  InputPortWidth=3  IndexOptions=Index vector (dialog),Index vector (dialog)  Indices=[1,2],[1,2]  OutputSizes=1,1
  Transform Sensor Base : sm_lib/Frames and Transforms/Transform Sensor  MeasurementFrame=Base  RotationSequence=XYX  SenseAngle=off  SenseAxis=off  SenseQ=off  SenseR=on  SenseRotationSequence=off  SenseOmegaX=off  SenseOmegaY=off  SenseOmegaZ=on  SenseOmega=off  SenseQDot=off  SenseRDot=off  SenseRotationSequenceDot=off  SenseAlphaX=off  SenseAlphaY=off  SenseAlphaZ=off  SenseAlpha=off  SenseQDDot=off  SenseRDDot=off  SenseX=off  SenseY=off  SenseZ=off  SenseXYZ=off  SenseRad=on  SenseAzim=on  SenseDist=off  SenseInc=off  SenseXDot=off  SenseYDot=off  SenseZDot=off  SenseXYZDot=off  SenseRadDot=on  SenseAzimDot=on  SenseDistDot=off  SenseIncDot=off  SenseXDDot=off  SenseYDDot=off  SenseZDDot=off  SenseXYZDDot=off  SenseRadDDot=off  SenseAzimDDot=off  SenseDistDDot=off  SenseIncDDot=off
  F : PMIOPort  Side=Left
  B : PMIOPort  Port=2  Side=Left
  rad : Outport  VectorParamsAs1DForOutWhenUnconnected=off
  vrad : Outport  Port=2  VectorParamsAs1DForOutWhenUnconnected=off
  azm : Outport  Port=3  VectorParamsAs1DForOutWhenUnconnected=off
  R : Outport  Port=4  VectorParamsAs1DForOutWhenUnconnected=off
  wz : Outport  Port=5  VectorParamsAs1DForOutWhenUnconnected=off
  vazm : Outport  Port=6  VectorParamsAs1DForOutWhenUnconnected=off
  wires:
  PS-Simulink Converter9/1 -> vazm/1
  PS-Simulink Converter8/1 -> wz/1
  PS-Simulink Converter6/1 -> Selector/1
  Selector/1 -> R/1
  PS-Simulink Converter4/1 -> vrad/1
  PS-Simulink Converter5/1 -> rad/1
  PS-Simulink Converter1/1 -> azm/1
  connections:
  PS-Simulink Converter9/LConn1 -- Transform Sensor Base/RConn7
  PS-Simulink Converter8/LConn1 -- Transform Sensor Base/RConn3
  Transform Sensor Base/RConn1 -- F/RConn1
  Transform Sensor Base/LConn1 -- B/RConn1
  PS-Simulink Converter6/LConn1 -- Transform Sensor Base/RConn2
  PS-Simulink Converter1/LConn1 -- Transform Sensor Base/RConn5
  PS-Simulink Converter5/LConn1 -- Transform Sensor Base/RConn4
  PS-Simulink Converter4/LConn1 -- Transform Sensor Base/RConn6

== system Contact_Forces_Lib/2D/Circle to Circle Force Enabled/Sum ==
  FnxCirF : Inport
  FnyCirF : Inport  Port=2
  FnxCirB : Inport  Port=3
  FnyCirB : Inport  Port=4
  FfxCirF : Inport  Port=5
  FfyCirF : Inport  Port=6
  FfxCirB : Inport  Port=7
  FfyCirB : Inport  Port=8
  TzCirF : Inport  Port=9
  TzCirB : Inport  Port=10
  Simulink-PS Converter{,3..7} (6 alike) : nesl_utility/Simulink-PS Converter  PhysicalDomain=network_engine_domain  SubClassName=ps_input  LeftPortType=input  RightPortType=output  PseudoPeriodic=off  Frequencies=[]  NoiseDistribution=none  NoiseParameters=[]  Unit=1  AffineConversion=off  FilteringAndDerivatives=zero  SimscapeFilterOrder=1  InputFilterTimeConstant=0.005  UdotUserProvided=[]
  Sum{2..5} (4 alike) : Sum
  FxF : PMIOPort  Side=Right
  FyF : PMIOPort  Port=2  Side=Right
  TzF : PMIOPort  Port=3  Side=Right
  FxB : PMIOPort  Port=4  Side=Right
  FyB : PMIOPort  Port=5  Side=Right
  TzB : PMIOPort  Port=6  Side=Right
  wires:
  Sum5/1 -> Simulink-PS Converter5/1
  Sum3/1 -> Simulink-PS Converter4/1
  Sum2/1 -> Simulink-PS Converter3/1
  Sum4/1 -> Simulink-PS Converter/1
  FnyCirB/1 -> Sum5/1
  FnxCirB/1 -> Sum3/1
  FnyCirF/1 -> Sum2/1
  FnxCirF/1 -> Sum4/1
  TzCirB/1 -> Simulink-PS Converter7/1
  TzCirF/1 -> Simulink-PS Converter6/1
  FfxCirB/1 -> Sum3/2
  FfyCirB/1 -> Sum5/2
  FfyCirF/1 -> Sum2/2
  FfxCirF/1 -> Sum4/2
  connections:
  Simulink-PS Converter7/RConn1 -- TzB/RConn1
  Simulink-PS Converter6/RConn1 -- TzF/RConn1
  Simulink-PS Converter5/RConn1 -- FyB/RConn1
  Simulink-PS Converter4/RConn1 -- FxB/RConn1
  Simulink-PS Converter3/RConn1 -- FyF/RConn1
  Simulink-PS Converter/RConn1 -- FxF/RConn1

== system Contact_Forces_Lib/2D/Circle to Finite Line Force/Calculate Penetration ==
  x : Inport
  vx : Inport  Port=2
  Abs : Abs  ZeroCross=off  SaturateOnIntegerOverflow=off
  Constant : Constant  Value=circle_rad+line_depth
  Dead Zone : DeadZone  LowerValue=-inf  UpperValue=0
  Gain2 : Gain  Gain=-1
  Product : Product
  Sign vx : Signum  ZeroCross=off
  Sign x : Signum  ZeroCross=off
  Sum : Sum  Inputs=+-
  Pos Sign : Outport  VectorParamsAs1DForOutWhenUnconnected=off
  Pen : Outport  Port=2  VectorParamsAs1DForOutWhenUnconnected=off
  Pen Vel : Outport  Port=3  VectorParamsAs1DForOutWhenUnconnected=off
  Vel Sign : Outport  Port=4  VectorParamsAs1DForOutWhenUnconnected=off
  wires:
  Gain2/1 -> Pen Vel/1
  Dead Zone/1 -> Pen/1
  Product/1 -> Gain2/1
  Sign vx/1 -> Vel Sign/1
  Sign x/1 -> Product/1, Pos Sign/1
  Abs/1 -> Sum/2
  Sum/1 -> Dead Zone/1
  Constant/1 -> Sum/1
  vx/1 -> Sign vx/1, Product/2
  x/1 -> Abs/1, Sign x/1

== system Contact_Forces_Lib/2D/Circle to Finite Line Force/Demux ==
  F : Inport
  Bus Creator : BusCreator  Inputs=2
  Bus Creator1 : BusCreator  Inputs=3
  Constant : Constant  Value=0
  Demux : Demux  Outputs=[3 3]
  Demux1 : Demux  Outputs=3
  Demux2 : Demux  Outputs=3
  Gain : Gain  Gain=-1
  Gain1 : Gain
  Simulink-PS Converter{,1..7} (8 alike) : nesl_utility/Simulink-PS Converter  PhysicalDomain=network_engine_domain  SubClassName=ps_input  LeftPortType=input  RightPortType=output  PseudoPeriodic=off  Frequencies=[]  NoiseDistribution=none  NoiseParameters=[]  Unit=1  AffineConversion=off  FilteringAndDerivatives=zero  SimscapeFilterOrder=1  InputFilterTimeConstant=0.005  UdotUserProvided=[]
  Fx Cir : PMIOPort  Side=Right
  Fy Cir : PMIOPort  Port=2  Side=Right
  Fz Cir : PMIOPort  Port=3  Side=Right
  Tz Cir : PMIOPort  Port=4  Side=Right
  Fx Lin : PMIOPort  Port=5  Side=Right
  Fy Lin : PMIOPort  Port=6  Side=Right
  Fz Lin : PMIOPort  Port=7  Side=Right
  Tz Lin : PMIOPort  Port=8  Side=Right
  FCir : Outport  VectorParamsAs1DForOutWhenUnconnected=off
  FLin : Outport  Port=2  VectorParamsAs1DForOutWhenUnconnected=off
  wires:
  Gain/1 -> Demux2/1
  Demux1/3 -> Simulink-PS Converter7/1
  Demux2/3 -> Bus Creator1/3, Simulink-PS Converter6/1  "Tz"
  Demux2/1 -> Bus Creator1/1, Simulink-PS Converter3/1  "Fx"
  Demux2/2 -> Bus Creator1/2, Simulink-PS Converter4/1  "Fy"
  Constant/1 -> Simulink-PS Converter5/1, Simulink-PS Converter2/1
  Demux1/2 -> Bus Creator/2, Simulink-PS Converter1/1  "Fy"
  Demux1/1 -> Bus Creator/1, Simulink-PS Converter/1  "Fx"
  Demux/1 -> Gain1/1
  Demux/2 -> Gain/1
  F/1 -> Demux/1
  Gain1/1 -> Demux1/1
  Bus Creator/1 -> FCir/1  "FCir"
  Bus Creator1/1 -> FLin/1  "FLin"
  connections:
  Tz Cir/RConn1 -- Simulink-PS Converter7/RConn1
  Fz Lin/RConn1 -- Simulink-PS Converter5/RConn1
  Fy Lin/RConn1 -- Simulink-PS Converter4/RConn1
  Fx Lin/RConn1 -- Simulink-PS Converter3/RConn1
  Tz Lin/RConn1 -- Simulink-PS Converter6/RConn1
  Fx Cir/RConn1 -- Simulink-PS Converter/RConn1
  Fy Cir/RConn1 -- Simulink-PS Converter1/RConn1
  Fz Cir/RConn1 -- Simulink-PS Converter2/RConn1

== system Contact_Forces_Lib/2D/Circle to Finite Line Force/Enable Force ==
  y : Inport
  Abs1 : Abs  ZeroCross=off  SaturateOnIntegerOverflow=off
  Activation limit for contact force : Constant  Value=line_length/2
  Sum : Sum  Inputs=+-
  Enable : Outport  VectorParamsAs1DForOutWhenUnconnected=off
  wires:
  Sum/1 -> Enable/1
  Activation limit for contact force/1 -> Sum/1
  y/1 -> Abs1/1
  Abs1/1 -> Sum/2

== system Contact_Forces_Lib/2D/Circle to Finite Line Force/Forces ==
  M arm : Inport
  X Sep : Inport  Port=2
  Pos Cmp : Inport  Port=3
  Pen : Inport  Port=4
  Vel : Inport  Port=5
  Vel_Cmp : Inport  Port=6
  Unit Vector : Inport  Port=7
  vy : Inport  Port=8
  wz : Inport  Port=9
  Action Port : ActionPort
  Force Law : $bdroot/Force Law  SystemSampleTime=-1  LabelModeActiveChoice=Linear  VariantActivationTime=update diagram  EmptyChoice=off  PassThrough=off  PassThroughVariantControl=(default)  EmptyChoiceVariantControl=(default)  AllowFlexibleInterface=on  Latency=0  AutoFrameSizeCalculation=off
  Mux : Mux  Inputs=6
  Resolve Forces : Subsystem
  Subsystem : Subsystem
  Fnf : Outport  InitialOutput=[0]  VectorParamsAs1DForOutWhenUnconnected=off
  F : Outport  Port=2  VectorParamsAs1DForOutWhenUnconnected=off
  wires:
  X Sep/1 -> Resolve Forces/3(X Sep)
  Force Law/2 -> Resolve Forces/5(Damp Force Mag)
  Force Law/1 -> Resolve Forces/4(Spr Force Mag)
  Resolve Forces/3(Tz Cir) -> Mux/3
  vy/1 -> Resolve Forces/8(vy)
  wz/1 -> Resolve Forces/9(wz)
  Unit Vector/1 -> Resolve Forces/7(Unit Vector)
  Vel_Cmp/1 -> Resolve Forces/6(Vel Cmp)
  Mux/1 -> F/1
  Pos Cmp/1 -> Resolve Forces/2(Pos Cmp)
  M arm/1 -> Resolve Forces/1(Moment arm)
  Resolve Forces/2(Fy Cir) -> Mux/2
  Resolve Forces/1(Fx Cir) -> Mux/1
  Resolve Forces/6(Tz Lin) -> Mux/6
  Resolve Forces/5(Fy Lin) -> Mux/5
  Vel/1 -> Force Law/2
  Pen/1 -> Force Law/1
  Resolve Forces/4(Fx Lin) -> Mux/4
  Resolve Forces/7(Fn) -> Subsystem/1(Fn)
  Resolve Forces/8(Ff) -> Subsystem/2(Ff)
  Subsystem/1(Out) -> Fnf/1

== system Contact_Forces_Lib/2D/Circle to Finite Line Force/No Force ==
  Action Port : ActionPort
  Zeros : Constant  Value=[0 0 0 0 0 0]  SampleTime=0
  Zeros1 : Constant  Value=[0 0]  SampleTime=0
  Fnf : Outport  InitialOutput=[0]  VectorParamsAs1DForOutWhenUnconnected=off
  F : Outport  Port=2  InitialOutput=[0 0 0 0 0 0]  VectorParamsAs1DForOutWhenUnconnected=off
  wires:
  Zeros/1 -> F/1
  Zeros1/1 -> Fnf/1

== system Contact_Forces_Lib/2D/Circle to Finite Line Force/Sensing ==
  PS-Simulink Converter{,1..5} (6 alike) : nesl_utility/PS-Simulink Converter  PhysicalDomain=network_engine_domain  SubClassName=ps_output  LeftPortType=input  RightPortType=output  PseudoPeriodic=off  Frequencies=[]  VectorFormat=1-D array  Unit=1  AffineConversion=off
  Selector : Selector  NumberOfDimensions=2  InputPortWidth=3  IndexOptions=Index vector (dialog),Index vector (dialog)  Indices=[1],[1,2]  OutputSizes=1,1
  Transform Sensor : sm_lib/Frames and Transforms/Transform Sensor  MeasurementFrame=Base  RotationSequence=XYX  SenseAngle=off  SenseAxis=off  SenseQ=off  SenseR=on  SenseRotationSequence=off  SenseOmegaX=off  SenseOmegaY=off  SenseOmegaZ=on  SenseOmega=off  SenseQDot=off  SenseRDot=off  SenseRotationSequenceDot=off  SenseAlphaX=off  SenseAlphaY=off  SenseAlphaZ=off  SenseAlpha=off  SenseQDDot=off  SenseRDDot=off  SenseX=on  SenseY=on  SenseZ=off  SenseXYZ=off  SenseRad=off  SenseAzim=off  SenseDist=off  SenseInc=off  SenseXDot=on  SenseYDot=on  SenseZDot=off  SenseXYZDot=off  SenseRadDot=off  SenseAzimDot=off  SenseDistDot=off  SenseIncDot=off  SenseXDDot=off  SenseYDDot=off  SenseZDDot=off  SenseXYZDDot=off  SenseRadDDot=off  SenseAzimDDot=off  SenseDistDDot=off  SenseIncDDot=off
  F : PMIOPort  Side=Left
  B : PMIOPort  Port=2  Side=Left
  y : Outport  VectorParamsAs1DForOutWhenUnconnected=off
  x : Outport  Port=2  VectorParamsAs1DForOutWhenUnconnected=off
  vx : Outport  Port=3  VectorParamsAs1DForOutWhenUnconnected=off
  q : Outport  Port=4  VectorParamsAs1DForOutWhenUnconnected=off
  vy : Outport  Port=5  VectorParamsAs1DForOutWhenUnconnected=off
  wz : Outport  Port=6  VectorParamsAs1DForOutWhenUnconnected=off
  wires:
  Selector/1 -> q/1
  PS-Simulink Converter5/1 -> Selector/1
  PS-Simulink Converter4/1 -> wz/1
  PS-Simulink Converter3/1 -> vy/1
  PS-Simulink Converter2/1 -> vx/1
  PS-Simulink Converter1/1 -> y/1
  PS-Simulink Converter/1 -> x/1
  connections:
  PS-Simulink Converter5/LConn1 -- Transform Sensor/RConn2
  PS-Simulink Converter3/LConn1 -- Transform Sensor/RConn7
  PS-Simulink Converter2/LConn1 -- Transform Sensor/RConn6
  PS-Simulink Converter1/LConn1 -- Transform Sensor/RConn5
  PS-Simulink Converter/LConn1 -- Transform Sensor/RConn4
  PS-Simulink Converter4/LConn1 -- Transform Sensor/RConn3
  Transform Sensor/LConn1 -- B/RConn1
  Transform Sensor/RConn1 -- F/RConn1

== system Contact_Forces_Lib/2D/Circle to Finite Line Force Enabled/Calculate Penetration ==
  x : Inport
  vx : Inport  Port=2
  Abs : Abs  ZeroCross=off  SaturateOnIntegerOverflow=off
  Constant : Constant  Value=circle_rad+line_depth
  Dead Zone : DeadZone  LowerValue=-inf  UpperValue=0
  Gain2 : Gain  Gain=-1
  Product : Product
  Sign vx : Signum  ZeroCross=off
  Sign x : Signum  ZeroCross=off
  Sum : Sum  Inputs=+-
  Pos Sign : Outport  VectorParamsAs1DForOutWhenUnconnected=off
  Pen : Outport  Port=2  VectorParamsAs1DForOutWhenUnconnected=off
  Pen Vel : Outport  Port=3  VectorParamsAs1DForOutWhenUnconnected=off
  Vel Sign : Outport  Port=4  VectorParamsAs1DForOutWhenUnconnected=off
  wires:
  x/1 -> Sign x/1, Abs/1
  vx/1 -> Product/2, Sign vx/1
  Constant/1 -> Sum/1
  Sum/1 -> Dead Zone/1
  Abs/1 -> Sum/2
  Sign x/1 -> Pos Sign/1, Product/1
  Sign vx/1 -> Vel Sign/1
  Product/1 -> Gain2/1
  Dead Zone/1 -> Pen/1
  Gain2/1 -> Pen Vel/1
